simulink model "BrakeController_Autosar"  (R2021b)
settings: Solver=FixedStepAuto  StartTime=0.0  StopTime=10.0  FixedStep=Ts  RelTol=1e-3
model workspace (MAT data in the model file):
  BrakePressure_Max = Simulink.Parameter
  BrakePressure_Max.Value = 100
  BrakePressure_Max.DataType = 'auto'
  BrakePressure_Max.Complexity = 'real'
  BrakePressure_Max.Dimensions = [1 1]
  Ts = Simulink.Parameter
  Ts.Value = 0.01
  Ts.DataType = 'auto'
  Ts.Complexity = 'real'
  Ts.Dimensions = [1 1]
  k = Simulink.Parameter
  k.Value = 2
  k.DataType = 'auto'
  k.Complexity = 'real'
  k.Dimensions = [1 1]
settings Model: Creator=QNH2KOR  LastModifiedBy=QNH2KOR
settings OptimizationCC: DefaultParameterBehavior=Inlined  EnhancedBackFolding=on  PassReuseOutputArgsAs=Individual arguments  ZeroExternalMemoryAtStartup=off  ZeroInternalMemoryAtStartup=off  OptimizeBlockOrder=speed  DifferentSizesBufferReuse=on  OptimizationCustomize=off  EfficientTunableParamExpr=on
settings DebuggingCC: ParameterTunabilityLossMsg=error
settings SFSimCC: MATLABDynamicMemAlloc=off
settings RTWCC: Description=AUTOSAR  SystemTargetFile=autosar.tlc  GenCodeOnly=on  TemplateMakefile=ert_default_tmf
settings CodeAppCC: ForceParamTrailComments=on  IgnoreCustomStorageClasses=off  OperatorAnnotations=on  SimulinkDataObjDesc=on  SFDataObjDesc=on  InsertBlockDesc=on
settings STFCustomTargetCC: TargetLangStandard=C99 (ISO)  MultiwordLength=256  ParMdlRefBuildCompliant=on  CompOptLevelCompliant=on  IncludeMdlTerminateFcn=off  CombineOutputUpdateFcns=on  SuppressErrorStatus=on  ERTCustomFileBanners=on  SupportNonFinite=off  SupportComplex=off  SupportContinuousTime=off  SupportNonInlinedSFcns=off  RemoveResetFunc=on  MATLABClassNameForMDSCustomization=Simulink.SoftwareTarget.ERTCustomization  AutosarCompliant=on  GRTInterface=off  UseToolchainInfoCompliant=on  LookupTableObjectStructAxisOrder=2,1,3,4,...  LUTObjectStructOrderEvenSpacing=Size,Table,Breakpoints  SystemTargetFile=autosar.tlc
settings ERTTargetCC: TargetLangStandard=C99 (ISO)  ConcurrentExecutionCompliant=off  IncludeMdlTerminateFcn=off  SuppressErrorStatus=on  SupportNonFinite=off  SupportComplex=off  ModelStepFunctionPrototypeControlCompliant=off  CPPClassGenCompliant=off  AutosarCompliant=on  LookupTableObjectStructAxisOrder=2,1,3,4,...  LUTObjectStructOrderEvenSpacing=Size,Table,Breakpoints  InlinedParameterPlacement=NonHierarchical  ERTCustomFileTemplate=example_file_process.tlc

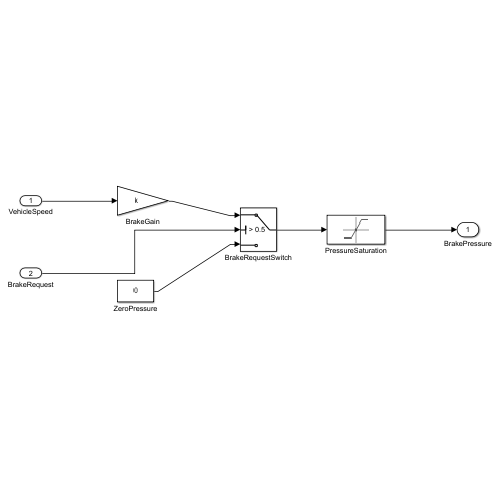
[thumbnail: Simulink's stored preview of the top-level diagram]
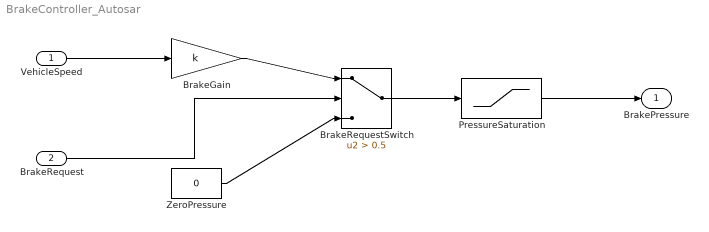
== system BrakeController_Autosar ==
  VehicleSpeed : Inport
  BrakeRequest : Inport  Port=2
  BrakeGain : Gain  Gain=k
  BrakeRequestSwitch : Switch  Criteria=u2 > Threshold  Threshold=0.5
  PressureSaturation : Saturate  UpperLimit=BrakePressure_Max  LowerLimit=0
  ZeroPressure : Constant  Value=0
  BrakePressure : Outport
  wires:
  VehicleSpeed/1 -> BrakeGain/1
  BrakeGain/1 -> BrakeRequestSwitch/1
  BrakeRequest/1 -> BrakeRequestSwitch/2
  ZeroPressure/1 -> BrakeRequestSwitch/3
  BrakeRequestSwitch/1 -> PressureSaturation/1
  PressureSaturation/1 -> BrakePressure/1
